simulink model "SistemaOriginal"  (R2026b)
settings: Solver=VariableStepAuto
values from neighbouring files (symbols this model uses):
  dtheta_init = 0    [Pendulo_Invertido.m]
  dx_init = 0    [Pendulo_Invertido.m]
  g = 9.80665    [Pendulo_Invertido.m]
  l = 0.30    (= 0.3)    [Pendulo_Invertido.m]
  M = m1+m2    (= 0.7)    [Pendulo_Invertido.m]
  m2 = 0.20    (= 0.2)    [Pendulo_Invertido.m]
  theta_init = pi - 20 * pi/180    (= 2.79252680319)    [Pendulo_Invertido.m]
  x_init = -0.35    [Pendulo_Invertido.m]
undefined symbols (not defined in the file or in its folder): c_theta, J
settings Model: Creator=fedeb  LastModifiedBy=fedeb

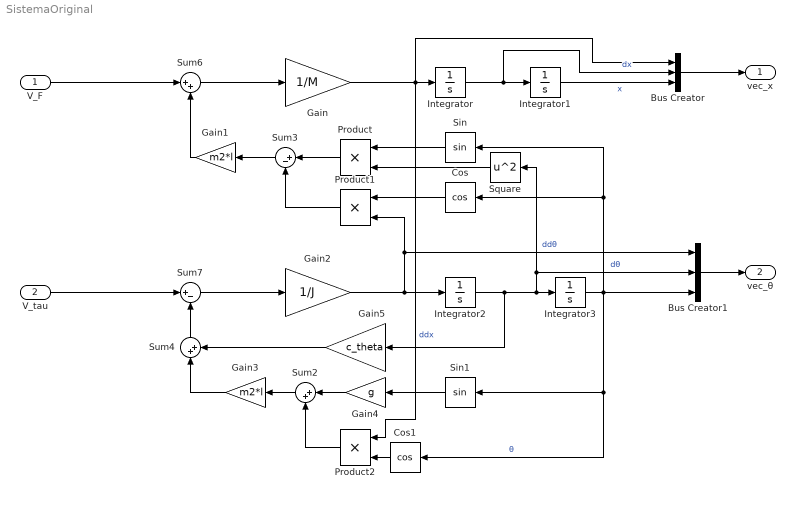
== system SistemaOriginal ==
  V_F : Inport
  V_tau : Inport  Port=2
  Bus Creator : BusCreator  Inputs=3
  Bus Creator1 : BusCreator  Inputs=3
  Cos : Trigonometry  Operator=cos
  Cos1 : Trigonometry  Operator=cos
  Gain : Gain  Gain=1/M
  Gain1 : Gain  Gain=m2*l
  Gain2 : Gain  Gain=1/J
  Gain3 : Gain  Gain=m2*l
  Gain4 : Gain  Gain=g
  Gain5 : Gain  Gain=c_theta
  Integrator : Integrator  InitialCondition=dx_init
  Integrator1 : Integrator  InitialCondition=x_init
  Integrator2 : Integrator  InitialCondition=dtheta_init
  Integrator3 : Integrator  InitialCondition=theta_init
  Product : Product
  Product1 : Product
  Product2 : Product
  Sin : Trigonometry
  Sin1 : Trigonometry
  Square : Math  Operator=square
  Sum2 : Sum  Inputs=|++
  Sum3 : Sum  Inputs=|+-
  Sum4 : Sum  Inputs=|++
  Sum6 : Sum  Inputs=|++
  Sum7 : Sum  Inputs=|+-
  vec_x : Outport
  vec_θ : Outport  Port=2
  wires:
  Sum6/1 -> Gain/1
  Gain/1 -> Bus Creator/1, Product2/1, Integrator/1  "ddx"
  Integrator/1 -> Bus Creator/2, Integrator1/1  "dx"
  Gain1/1 -> Sum6/2
  Integrator2/1 -> Gain5/1, Bus Creator1/2, Square/1, Integrator3/1  "dθ"
  Sum7/1 -> Gain2/1
  Gain2/1 -> Bus Creator1/1, Product1/2, Integrator2/1  "ddθ"
  Integrator3/1 -> Cos/1, Sin/1, Bus Creator1/3, Sin1/1, Cos1/1  "θ"
  V_tau/1 -> Sum7/1
  Sin/1 -> Product/1
  Sum3/1 -> Gain1/1
  Product/1 -> Sum3/1
  Cos/1 -> Product1/1
  Cos1/1 -> Product2/2
  Sum2/1 -> Gain3/1
  Product2/1 -> Sum2/2
  Gain4/1 -> Sum2/1
  Sin1/1 -> Gain4/1
  Sum4/1 -> Sum7/2
  Gain3/1 -> Sum4/1
  Gain5/1 -> Sum4/2
  Square/1 -> Product/2
  Integrator1/1 -> Bus Creator/3  "x"
  Bus Creator/1 -> vec_x/1
  Bus Creator1/1 -> vec_θ/1
  Product1/1 -> Sum3/2
  V_F/1 -> Sum6/1
